simulink model "q_current_controller_discrete"  (R2025b)
settings: Solver=FixedStepDiscrete  FixedStep=control.currentLoopPeriod_s
undefined symbols (not defined in the file): control, DiscIntNeverNeededParam
settings Model: Creator=semih  LastModifiedBy=Semih
settings SFSimCC: SimGPUStackLimitPerThread=51200  SimGPUMallocThreshold=200
settings RTWCC: GPUStackLimitPerThread=51200  GPUMallocThreshold=200
settings GRTTargetCC: CombineOutputUpdateFcns=off

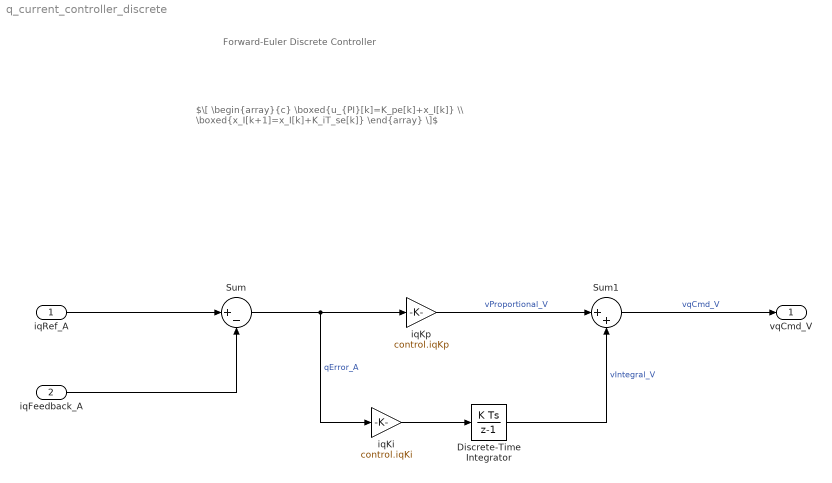
== system q_current_controller_discrete ==
  note: Forward-Euler Discrete Controller
  note: $\[ \begin{array}{c} \boxed{u_{PI}[k]=K_pe[k]+x_I[k]} \\ \boxed{x_I[k+1]=x_I[k]+K_iT_se[k]} \end{array} \]$
  iqRef_A : Inport
  iqFeedback_A : Inport  Port=2
  Discrete-Time Integrator : DiscreteIntegrator  SampleTime=control.currentLoopPeriod_s  ICPrevOutput=DiscIntNeverNeededParam  ICPrevScaledInput=DiscIntNeverNeededParam
  Sum : Sum  Inputs=|+-
  Sum1 : Sum  Inputs=|++
  iqKi : Gain  Gain=control.iqKi
  iqKp : Gain  Gain=control.iqKp
  vqCmd_V : Outport
  wires:
  iqRef_A/1 -> Sum/1
  iqFeedback_A/1 -> Sum/2
  Sum/1 -> iqKp/1, iqKi/1  "qError_A"
  iqKi/1 -> Discrete-Time Integrator/1
  Sum1/1 -> vqCmd_V/1  "vqCmd_V"
  iqKp/1 -> Sum1/1  "vProportional_V"
  Discrete-Time Integrator/1 -> Sum1/2  "vIntegral_V"
